simulink model "wrist_model"  (R2026a)
settings: Solver=VariableStepAuto  StopTime=2  MaxStep=0.02
undefined symbols (not defined in the file or in its folder): Kp_motor_angle, R_motor_gearbox
settings Model: Creator=ander  LastModifiedBy=ander

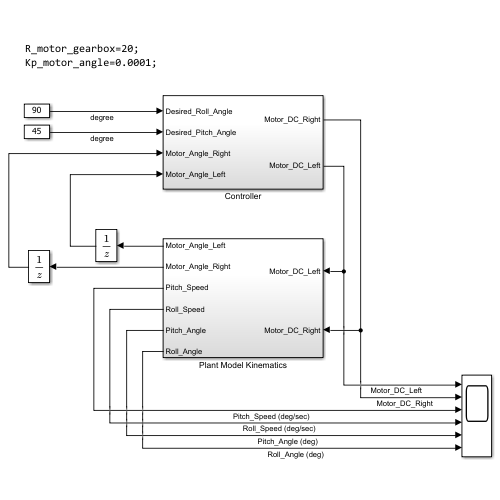
[thumbnail: Simulink's stored preview of the top-level diagram]
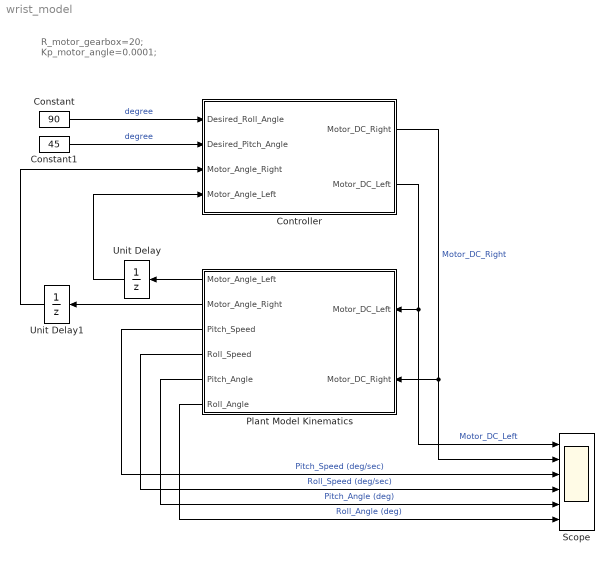
== system wrist_model ==
  note: R_motor_gearbox=20;
      | Kp_motor_angle=0.0001;
  Constant : Constant  Value=90
  Constant1 : Constant  Value=45
  Controller : Subsystem
  Plant Model Kinematics : Subsystem
  Scope : Scope  NumInputPorts=6
      settings: ActiveDisplayYMinimum=-0.033652419375443353  ActiveDisplayYMaximum=0.30373915770838261
  Unit Delay : UnitDelay  SampleTime=0.02
  Unit Delay1 : UnitDelay  SampleTime=0.02
  wires:
  Controller/2(Motor_DC_Left) -> Scope/1, Plant Model Kinematics/1(Motor_DC_Left)  "Motor_DC_Left"
  Controller/1(Motor_DC_Right) -> Scope/2, Plant Model Kinematics/2(Motor_DC_Right)  "Motor_DC_Right"
  Constant/1 -> Controller/1(Desired_Roll_Angle)  "degree"
  Constant1/1 -> Controller/2(Desired_Pitch_Angle)  "degree"
  Plant Model Kinematics/1(Motor_Angle_Left) -> Unit Delay/1
  Plant Model Kinematics/2(Motor_Angle_Right) -> Unit Delay1/1
  Plant Model Kinematics/3(Pitch_Speed) -> Scope/3  "Pitch_Speed (deg/sec)"
  Plant Model Kinematics/4(Roll_Speed) -> Scope/4  "Roll_Speed (deg/sec)"
  Plant Model Kinematics/5(Pitch_Angle) -> Scope/5  "Pitch_Angle (deg)"
  Plant Model Kinematics/6(Roll_Angle) -> Scope/6  "Roll_Angle (deg)"
  Unit Delay/1 -> Controller/4(Motor_Angle_Left)
  Unit Delay1/1 -> Controller/3(Motor_Angle_Right)

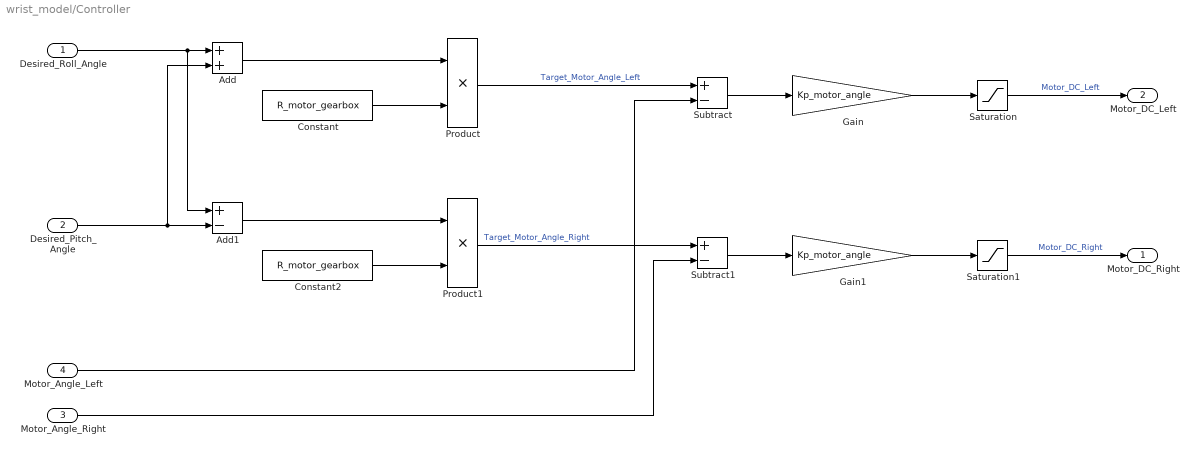
== system wrist_model/Controller ==
  Desired_Roll_Angle : Inport
  Desired_Pitch_Angle : Inport  Port=2
  Motor_Angle_Right : Inport  Port=3
  Motor_Angle_Left : Inport  Port=4
  Add : Sum
  Add1 : Sum  Inputs=+-
  Constant : Constant  Value=R_motor_gearbox
  Constant2 : Constant  Value=R_motor_gearbox
  Gain : Gain  Gain=Kp_motor_angle
  Gain1 : Gain  Gain=Kp_motor_angle
  Product : Product  Inputs=**
  Product1 : Product  Inputs=**
  Saturation : Saturate  UpperLimit=1  LowerLimit=-1
  Saturation1 : Saturate  UpperLimit=1  LowerLimit=-1
  Subtract : Sum  Inputs=+-
  Subtract1 : Sum  Inputs=+-
  Motor_DC_Right : Outport
  Motor_DC_Left : Outport  Port=2
  wires:
  Desired_Roll_Angle/1 -> Add1/1, Add/1
  Desired_Pitch_Angle/1 -> Add/2, Add1/2
  Add/1 -> Product/1
  Constant/1 -> Product/2
  Product/1 -> Subtract/1  "Target_Motor_Angle_Left"
  Constant2/1 -> Product1/2
  Add1/1 -> Product1/1
  Product1/1 -> Subtract1/1  "Target_Motor_Angle_Right"
  Motor_Angle_Left/1 -> Subtract/2
  Motor_Angle_Right/1 -> Subtract1/2
  Subtract/1 -> Gain/1
  Subtract1/1 -> Gain1/1
  Gain/1 -> Saturation/1
  Gain1/1 -> Saturation1/1
  Saturation/1 -> Motor_DC_Left/1  "Motor_DC_Left"
  Saturation1/1 -> Motor_DC_Right/1  "Motor_DC_Right"

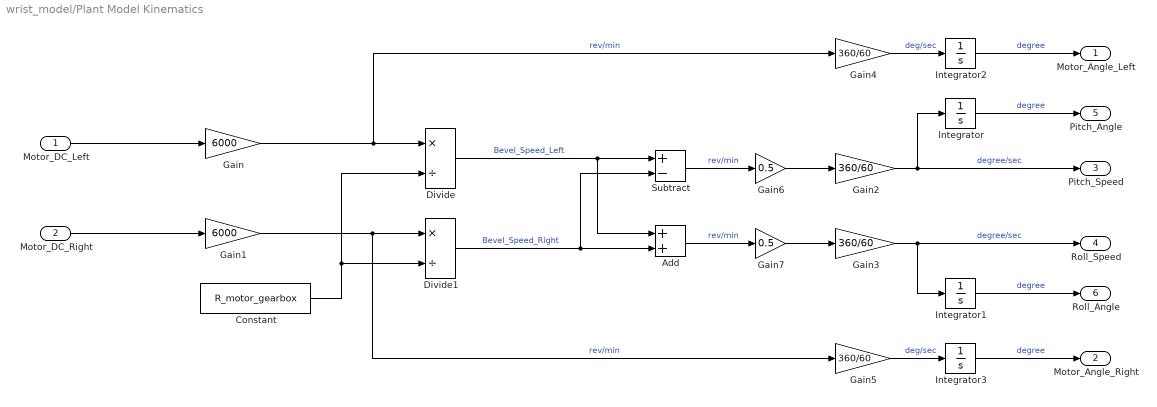
== system wrist_model/Plant Model Kinematics ==
  Motor_DC_Left : Inport
  Motor_DC_Right : Inport  Port=2
  Add : Sum
  Constant : Constant  Value=R_motor_gearbox
  Divide : Product  Inputs=*/
  Divide1 : Product  Inputs=*/
  Gain : Gain  Gain=6000
  Gain1 : Gain  Gain=6000
  Gain{2..5} (4 alike) : Gain  Gain=360/60
  Gain6 : Gain  Gain=0.5
  Gain7 : Gain  Gain=0.5
  Integrator{,1..3} (4 alike) : Integrator
  Subtract : Sum  Inputs=+-
  Motor_Angle_Left : Outport
  Motor_Angle_Right : Outport  Port=2
  Pitch_Speed : Outport  Port=3
  Roll_Speed : Outport  Port=4
  Pitch_Angle : Outport  Port=5
  Roll_Angle : Outport  Port=6
  wires:
  Divide/1 -> Add/1, Subtract/1  "Bevel_Speed_Left"
  Divide1/1 -> Add/2, Subtract/2  "Bevel_Speed_Right"
  Subtract/1 -> Gain6/1  "rev/min"
  Add/1 -> Gain7/1  "rev/min"
  Gain2/1 -> Integrator/1, Pitch_Speed/1  "degree/sec"
  Gain3/1 -> Integrator1/1, Roll_Speed/1  "degree/sec"
  Integrator/1 -> Pitch_Angle/1  "degree"
  Integrator1/1 -> Roll_Angle/1  "degree"
  Constant/1 -> Divide1/2, Divide/2
  Integrator2/1 -> Motor_Angle_Left/1  "degree"
  Integrator3/1 -> Motor_Angle_Right/1  "degree"
  Gain/1 -> Gain4/1, Divide/1  "rev/min"
  Gain1/1 -> Gain5/1, Divide1/1  "rev/min"
  Gain4/1 -> Integrator2/1  "deg/sec"
  Gain5/1 -> Integrator3/1  "deg/sec"
  Motor_DC_Left/1 -> Gain/1
  Motor_DC_Right/1 -> Gain1/1
  Gain6/1 -> Gain2/1
  Gain7/1 -> Gain3/1
